simulink model "Hopper_GMEKF_Simulation"  (R2026a)
settings: Solver=FixedStepDiscrete  StartTime=0  StopTime=10  FixedStep=0.002
undefined symbols (not defined in the file or in its folder): barometer_st, gps_frame, gps_st, imu_st, lidar_frames, lidar_st, qc
settings Model: DataDictionary=NavigationDictionary.sldd  Creator=David  LastModifiedBy=David

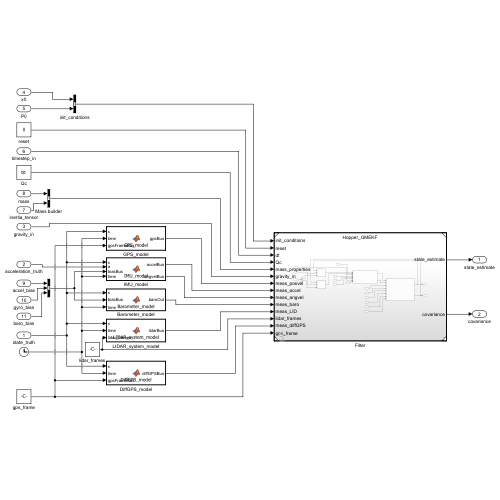
[thumbnail: Simulink's stored preview of the top-level diagram]
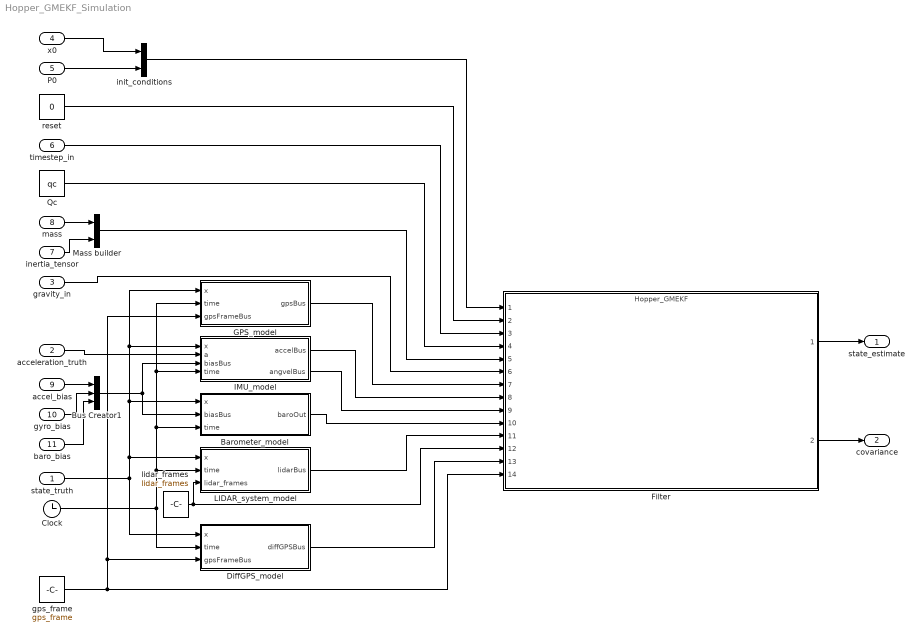
== system Hopper_GMEKF_Simulation ==
  state_truth : Inport  PortDimensions=[20 1]
  acceleration_truth : Inport  Port=2  PortDimensions=[3 1]
  gravity_in : Inport  Port=3  PortDimensions=1
  x0 : Inport  Port=4  PortDimensions=[20 1]
  P0 : Inport  Port=5  PortDimensions=[19 19]
  timestep_in : Inport  Port=6
  inertia_tensor : Inport  Port=7  PortDimensions=[3 3]
  mass : Inport  Port=8  PortDimensions=1
  accel_bias : Inport  Port=9  PortDimensions=[3 1]
  gyro_bias : Inport  Port=10  PortDimensions=[3 1]
  baro_bias : Inport  Port=11  PortDimensions=1
  Barometer_model : MATLAB Function  TreatAsAtomicUnit=on  SystemSampleTime=barometer_st
  Bus Creator1 : BusCreator  Inputs=3  OutDataTypeStr=Bus: biasBus
      settings: InheritFromInputs=off
  Clock : Clock
  DiffGPS_model : MATLAB Function  TreatAsAtomicUnit=on  SystemSampleTime=gps_st
  Filter : ModelReference  ModelNameDialog=Hopper_GMEKF.slx  SimulationMode=Normal  ModelReferenceVersion=1.59
  GPS_model : MATLAB Function  TreatAsAtomicUnit=on  SystemSampleTime=gps_st
  IMU_model : MATLAB Function  TreatAsAtomicUnit=on  SystemSampleTime=imu_st
  LIDAR_system_model : MATLAB Function  TreatAsAtomicUnit=on  SystemSampleTime=lidar_st
  Mass builder : BusCreator  Inputs=2  OutDataTypeStr=Bus: massProperties
      settings: InheritFromInputs=off
  Qc : Constant  Value=qc  OutDataTypeStr=ValueType: Qc
  gps_frame : Constant  Value=gps_frame  OutDataTypeStr=Bus: gpsFrameBus
  init_conditions : BusCreator  Inputs=2  OutDataTypeStr=Bus: InitConditions
      settings: InheritFromInputs=off
  lidar_frames : Constant  Value=lidar_frames  OutDataTypeStr=Bus: lidarFrameBus
  reset : Constant  Value=0
  state_estimate : Outport  PortDimensions=[20 1]
  covariance : Outport  Port=2  PortDimensions=[19 19]
  wires:
  Filter/1 -> state_estimate/1
  Filter/2 -> covariance/1
  state_truth/1 -> GPS_model/1(x), IMU_model/1(x), Barometer_model/1(x), LIDAR_system_model/1(x), DiffGPS_model/1(x)
  acceleration_truth/1 -> IMU_model/2(a)
  Clock/1 -> GPS_model/2(time), IMU_model/4(time), Barometer_model/3(time), LIDAR_system_model/2(time), DiffGPS_model/2(time)
  P0/1 -> init_conditions/2
  x0/1 -> init_conditions/1
  init_conditions/1 -> Filter/1
  Bus Creator1/1 -> Barometer_model/2(biasBus), IMU_model/3(biasBus)
  reset/1 -> Filter/2
  timestep_in/1 -> Filter/3
  gravity_in/1 -> Filter/6
  Qc/1 -> Filter/4
  lidar_frames/1 -> Filter/12, LIDAR_system_model/3(lidar_frames)
  gps_frame/1 -> Filter/14, DiffGPS_model/3(gpsFrameBus), GPS_model/3(gpsFrameBus)
  mass/1 -> Mass builder/1
  inertia_tensor/1 -> Mass builder/2
  Mass builder/1 -> Filter/5
  accel_bias/1 -> Bus Creator1/1
  gyro_bias/1 -> Bus Creator1/2
  baro_bias/1 -> Bus Creator1/3
  GPS_model/1(gpsBus) -> Filter/7
  IMU_model/1(accelBus) -> Filter/8
  IMU_model/2(angvelBus) -> Filter/9
  Barometer_model/1(baroOut) -> Filter/10
  LIDAR_system_model/1(lidarBus) -> Filter/11
  DiffGPS_model/1(diffGPSBus) -> Filter/13

== matlab function Hopper_GMEKF_Simulation/IMU_model ==
  data: x input; accelBus output Bus: accelBus; angvelBus output Bus: angvelBus; a input; biasBus input; time input
function [accelBus, angvelBus] = IMU_model(x, a, biasBus, time)
ab = biasBus.accelBias;
gb = biasBus.gyroBias;
[accelBus, angvelBus] = imu_model(x, a, ab, gb, time);
end

== matlab function Hopper_GMEKF_Simulation/GPS_model ==
  data: x input size=[20 1]; gpsBus output Bus: gpsBus; time input; gpsFrameBus input
function gpsBus = GPS_model(x, time, gpsFrameBus)
gpsBus = gps_model(x, time, gpsFrameBus);
end

== matlab function Hopper_GMEKF_Simulation/Barometer_model ==
  data: x input; biasBus input; baroOut output Bus: baroBus; time input
function baroOut = Barometer_model(x, biasBus, time)
bb = biasBus.baroBias;
baroOut = barometer_model(x, bb, time);
end

== matlab function Hopper_GMEKF_Simulation/LIDAR_system_model ==
  data: x input; lidarBus output Bus: lidarBus; time input; lidar_frames input
function lidarBus = LIDAR_system_model(x, time, lidar_frames)
lidarBus = lidar_system_model(x, time, lidar_frames);
end

== matlab function Hopper_GMEKF_Simulation/DiffGPS_model ==
  data: x input; diffGPSBus output Bus: diffGpsBus; time input; gpsFrameBus input
function diffGPSBus = DiffGPS_model(x, time, gpsFrameBus)
diffGPSBus = diffGps_model(x, time, gpsFrameBus);
